simulink model "pid_analog_circuit"  (R2024b)
settings: Solver=ode4  StartTime=0.0  StopTime=1  FixedStep=pcb.sim_dt  RelTol=1e-3
PostLoadFcn:
  | pacdir_ = fileparts(get_param('pid_analog_circuit','FileName')); if ~exist('pcb','var'), run(fullfile(pacdir_,'pid_board_params.m')); end; if ~exist('pacirc','var'), run(fullfile(pacdir_,'pid_analog_circuit_params.m')); end; clear pacdir_
values from neighbouring files (symbols this model uses):
  pacirc = struct()    [pid_analog_circuit_params.m]
  pcb = evalin('base', 'pcb')    [pid_analog_circuit_test.m]    (also in pid_board_bench_inputs.m; pid_board_params.m = struct(); pid_board_validate.m)
libraries: ee_lib x153, fl_lib x61, nesl_utility x48
(part 1 of 5)
Description:
  | PID_Board rev B analog section, Simscape Electrical component-level model (circuit variant). Ports per ANALOG_INTERFACE.md. Params: pcb (pid_board_params.m) + pacirc (pid_analog_circuit_params.m).
settings Model: Creator=doubi  LastModifiedBy=doubi
settings DataIOCC: LoadExternalInput=on  SaveFormat=StructureWithTime

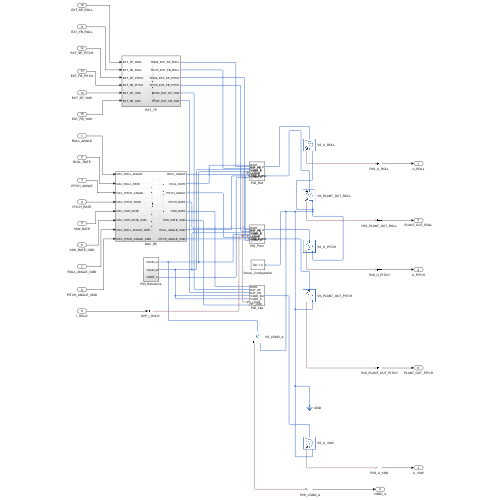
[thumbnail: Simulink's stored preview of the top-level diagram]
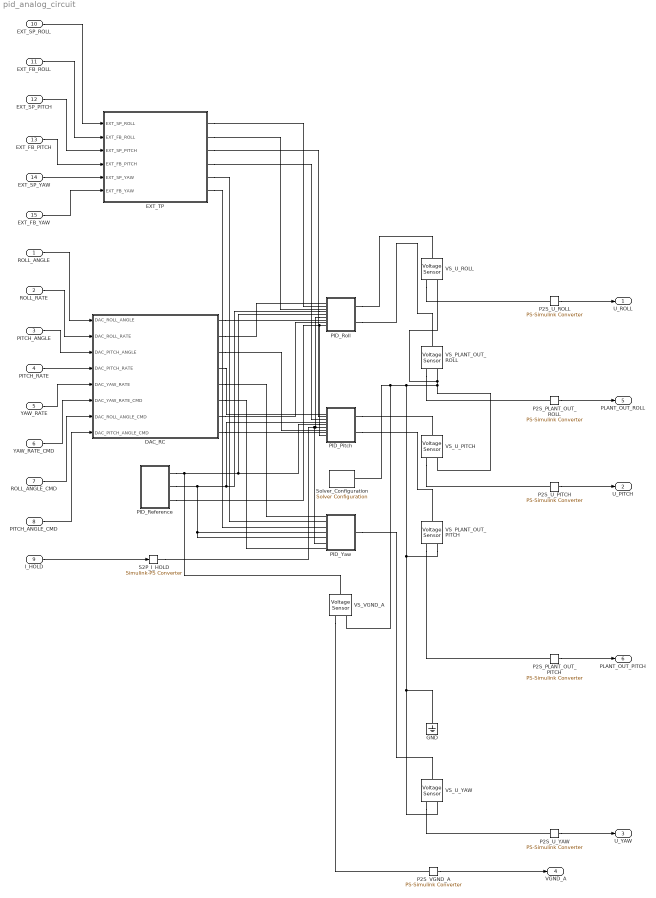
== system pid_analog_circuit ==
  ROLL_ANGLE : Inport
  ROLL_RATE : Inport  Port=2
  PITCH_ANGLE : Inport  Port=3
  PITCH_RATE : Inport  Port=4
  YAW_RATE : Inport  Port=5
  YAW_RATE_CMD : Inport  Port=6
  ROLL_ANGLE_CMD : Inport  Port=7
  PITCH_ANGLE_CMD : Inport  Port=8
  I_HOLD : Inport  Port=9
  EXT_SP_ROLL : Inport  Port=10
  EXT_FB_ROLL : Inport  Port=11
  EXT_SP_PITCH : Inport  Port=12
  EXT_FB_PITCH : Inport  Port=13
  EXT_SP_YAW : Inport  Port=14
  EXT_FB_YAW : Inport  Port=15
  DAC_RC : Subsystem
  EXT_TP : Subsystem
  GND : fl_lib/Electrical/Electrical Elements/Electrical Reference
  P2S_PLANT_OUT_PITCH : nesl_utility/PS-Simulink Converter  PhysicalDomain=network_engine_domain  SubClassName=ps_output  LeftPortType=input  RightPortType=output  PseudoPeriodic=off  Frequencies=[]  VectorFormat=inherit  Unit=V  AffineConversion=off
  P2S_PLANT_OUT_ROLL : nesl_utility/PS-Simulink Converter  PhysicalDomain=network_engine_domain  SubClassName=ps_output  LeftPortType=input  RightPortType=output  PseudoPeriodic=off  Frequencies=[]  VectorFormat=inherit  Unit=V  AffineConversion=off
  P2S_U_PITCH : nesl_utility/PS-Simulink Converter  PhysicalDomain=network_engine_domain  SubClassName=ps_output  LeftPortType=input  RightPortType=output  PseudoPeriodic=off  Frequencies=[]  VectorFormat=inherit  Unit=V  AffineConversion=off
  P2S_U_ROLL : nesl_utility/PS-Simulink Converter  PhysicalDomain=network_engine_domain  SubClassName=ps_output  LeftPortType=input  RightPortType=output  PseudoPeriodic=off  Frequencies=[]  VectorFormat=inherit  Unit=V  AffineConversion=off
  P2S_U_YAW : nesl_utility/PS-Simulink Converter  PhysicalDomain=network_engine_domain  SubClassName=ps_output  LeftPortType=input  RightPortType=output  PseudoPeriodic=off  Frequencies=[]  VectorFormat=inherit  Unit=V  AffineConversion=off
  P2S_VGND_A : nesl_utility/PS-Simulink Converter  PhysicalDomain=network_engine_domain  SubClassName=ps_output  LeftPortType=input  RightPortType=output  PseudoPeriodic=off  Frequencies=[]  VectorFormat=inherit  Unit=V  AffineConversion=off
  PID_Pitch : Subsystem  mask{ax=pcb.pitch}
      mask prompts: ax "Axis parameter struct (pcb.roll / pcb.pitch / pcb.yaw)"
      mask help: PID_Roll sheet (U201/U202, U9A): rate cell + angle loop + bench plant. Values from pcb.roll; part models from pacirc.
  PID_Reference : Subsystem
  PID_Roll : Subsystem  mask{ax=pcb.roll}
      mask prompts: ax "Axis parameter struct (pcb.roll / pcb.pitch / pcb.yaw)"
      mask help: PID_Roll sheet (U201/U202, U9A): rate cell + angle loop + bench plant. Values from pcb.roll; part models from pacirc.
  PID_Yaw : Subsystem  mask{ax=pcb.yaw}
      mask prompts: ax "Axis parameter struct (pcb.roll / pcb.pitch / pcb.yaw)"
      mask help: PID_Roll sheet (U201/U202, U9A): rate cell + angle loop + bench plant. Values from pcb.roll; part models from pacirc.
  S2P_I_HOLD : nesl_utility/Simulink-PS Converter  PhysicalDomain=network_engine_domain  SubClassName=ps_input  LeftPortType=input  RightPortType=output  PseudoPeriodic=off  Frequencies=[]  NoiseDistribution=none  NoiseParameters=[]  Unit=1  AffineConversion=off  FilteringAndDerivatives=provide  SimscapeFilterOrder=1  InputFilterTimeConstant=0.001  UdotUserProvided=0
  Solver_Configuration : nesl_utility/Solver Configuration  PhysicalDomain=network_engine_domain  SubClassName=solver  LeftPortType=input  RightPortType=generic  Tones=[]  Harmonics=[]  SimulateNoise=off  Profile=off  UseLocalSampling=off  EnableSwitchedLinearOptims=on  FrequencyDomain=off  UseCCode=off  RelTol=0.001  AbsTol=0.001  MinStep=1e-09  ToWorkspace=off  RevertToSquareIcSolve=off  NumHomotopyIterations=100  PhasorMode=off  PhasorModeNumHarmonics=1  ConsistencySolver=NEWTON_XTOL_AFTER_FTOL  IndexReductionMethod=DerivativeReplacement  DoDC=off  ResidualTolerance=1e-09  ConsistencyTolSource=GLOBAL  ConsistencyAbsTol=0.001  ConsistencyRelTol=0.001  ConsistencyTolFactor=0.001  UseLocalSolver=on  LocalSolverChoice=NE_BACKWARD_EULER_ADVANCER  ResolveIndetEquations=on  FunctionEvalNumThread=1  LocalSolverSampleTime=pacirc.Ts  DoFixedCost=on  MaxNonlinIter=pacirc.nl_iter  MaxModeIter=2  ComputeImpulses=off  ImpulseIterations=2  LinearAlgebra=auto  LinearAlgebraNumThread=0  EquationFormulation=NE_TIME_EF  DelaysMemoryBudget=1024  AutomaticFiltering=on  FilteringTimeConstant=0.001  PartitionStorageMethod=AS_NEEDED  PartitionMemoryBudget=1024  PartitionMethod=ROBUST  MultibodyUseLocalSolver=off  MultibodyLocalSolverChoice=ODE1  MultibodyLocalSolverSampleTime=0.001
  VS_PLANT_OUT_PITCH : fl_lib/Electrical/Electrical Sensors/Voltage Sensor
  VS_PLANT_OUT_ROLL : fl_lib/Electrical/Electrical Sensors/Voltage Sensor
  VS_U_PITCH : fl_lib/Electrical/Electrical Sensors/Voltage Sensor
  VS_U_ROLL : fl_lib/Electrical/Electrical Sensors/Voltage Sensor
  VS_U_YAW : fl_lib/Electrical/Electrical Sensors/Voltage Sensor
  VS_VGND_A : fl_lib/Electrical/Electrical Sensors/Voltage Sensor
  U_ROLL : Outport
  U_PITCH : Outport  Port=2
  U_YAW : Outport  Port=3
  VGND_A : Outport  Port=4
  PLANT_OUT_ROLL : Outport  Port=5
  PLANT_OUT_PITCH : Outport  Port=6
  wires:
  P2S_PLANT_OUT_PITCH/1 -> PLANT_OUT_PITCH/1
  P2S_PLANT_OUT_ROLL/1 -> PLANT_OUT_ROLL/1
  P2S_VGND_A/1 -> VGND_A/1
  P2S_U_YAW/1 -> U_YAW/1
  P2S_U_PITCH/1 -> U_PITCH/1
  P2S_U_ROLL/1 -> U_ROLL/1
  I_HOLD/1 -> S2P_I_HOLD/1
  EXT_FB_YAW/1 -> EXT_TP/6(EXT_FB_YAW)
  EXT_SP_YAW/1 -> EXT_TP/5(EXT_SP_YAW)
  EXT_FB_PITCH/1 -> EXT_TP/4(EXT_FB_PITCH)
  ROLL_ANGLE/1 -> DAC_RC/1(DAC_ROLL_ANGLE)
  ROLL_RATE/1 -> DAC_RC/2(DAC_ROLL_RATE)
  PITCH_ANGLE/1 -> DAC_RC/3(DAC_PITCH_ANGLE)
  PITCH_RATE/1 -> DAC_RC/4(DAC_PITCH_RATE)
  YAW_RATE/1 -> DAC_RC/5(DAC_YAW_RATE)
  YAW_RATE_CMD/1 -> DAC_RC/6(DAC_YAW_RATE_CMD)
  ROLL_ANGLE_CMD/1 -> DAC_RC/7(DAC_ROLL_ANGLE_CMD)
  PITCH_ANGLE_CMD/1 -> DAC_RC/8(DAC_PITCH_ANGLE_CMD)
  EXT_SP_ROLL/1 -> EXT_TP/1(EXT_SP_ROLL)
  EXT_FB_ROLL/1 -> EXT_TP/2(EXT_FB_ROLL)
  EXT_SP_PITCH/1 -> EXT_TP/3(EXT_SP_PITCH)
  connections:
  VS_PLANT_OUT_PITCH/RConn1 -- P2S_PLANT_OUT_PITCH/LConn1
  PID_Pitch/RConn2 -- VS_PLANT_OUT_PITCH/LConn1
  VS_PLANT_OUT_ROLL/RConn1 -- P2S_PLANT_OUT_ROLL/LConn1
  PID_Roll/RConn2 -- VS_PLANT_OUT_ROLL/LConn1
  VS_VGND_A/RConn1 -- P2S_VGND_A/LConn1
  VS_U_YAW/RConn1 -- P2S_U_YAW/LConn1
  PID_Yaw/RConn1 -- VS_U_YAW/LConn1
  VS_U_PITCH/RConn1 -- P2S_U_PITCH/LConn1
  PID_Pitch/RConn1 -- VS_U_PITCH/LConn1
  VS_U_ROLL/RConn1 -- P2S_U_ROLL/LConn1
  PID_Roll/RConn1 -- VS_U_ROLL/LConn1
  VS_PLANT_OUT_PITCH/RConn2 -- VS_U_YAW/RConn2 -- GND/LConn1 -- VS_VGND_A/RConn2 -- Solver_Configuration/RConn1 -- VS_PLANT_OUT_ROLL/RConn2 -- VS_U_ROLL/RConn2 -- VS_U_PITCH/RConn2
  EXT_TP/RConn6 -- PID_Yaw/LConn3
  EXT_TP/RConn5 -- PID_Yaw/LConn2
  EXT_TP/RConn4 -- PID_Pitch/LConn3
  EXT_TP/RConn3 -- PID_Pitch/LConn2
  EXT_TP/RConn2 -- PID_Roll/LConn3
  EXT_TP/RConn1 -- PID_Roll/LConn2
  DAC_RC/RConn8 -- PID_Pitch/LConn8
  DAC_RC/RConn7 -- PID_Roll/LConn8
  DAC_RC/RConn6 -- PID_Yaw/LConn7
  DAC_RC/RConn5 -- PID_Yaw/LConn1
  DAC_RC/RConn4 -- PID_Pitch/LConn1
  DAC_RC/RConn3 -- PID_Pitch/LConn7
  DAC_RC/RConn2 -- PID_Roll/LConn1
  DAC_RC/RConn1 -- PID_Roll/LConn7
  PID_Pitch/LConn9 -- PID_Reference/RConn3 -- PID_Roll/LConn9
  PID_Roll/LConn4 -- PID_Reference/RConn2 -- PID_Yaw/LConn4 -- PID_Yaw/LConn5 -- PID_Pitch/LConn4
  PID_Pitch/LConn5 -- PID_Reference/RConn1 -- VS_VGND_A/LConn1 -- PID_Roll/LConn5
  PID_Roll/LConn6 -- S2P_I_HOLD/RConn1 -- PID_Yaw/LConn6 -- PID_Pitch/LConn6

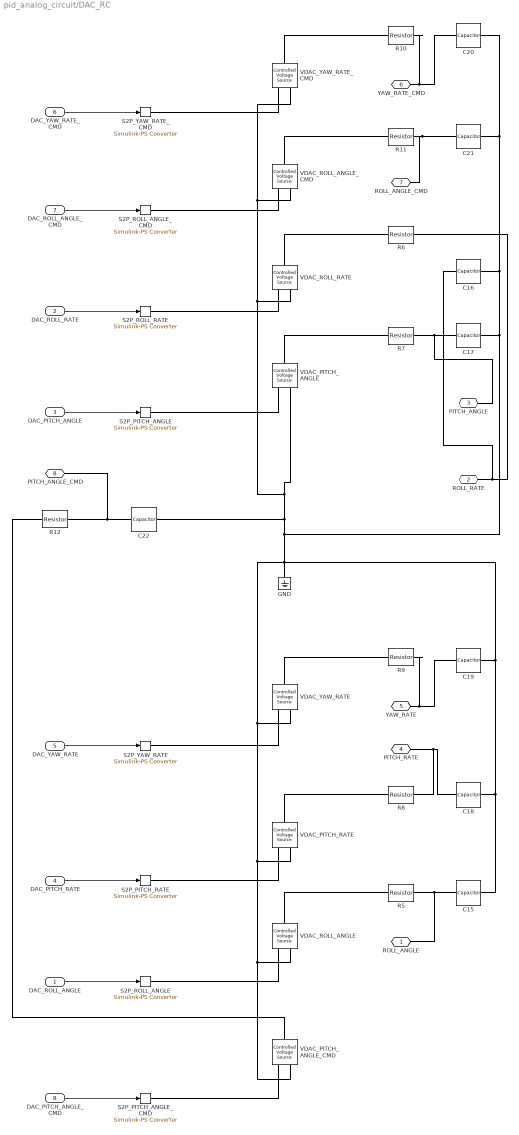
== system pid_analog_circuit/DAC_RC ==
  DAC_ROLL_ANGLE : Inport
  DAC_ROLL_RATE : Inport  Port=2
  DAC_PITCH_ANGLE : Inport  Port=3
  DAC_PITCH_RATE : Inport  Port=4
  DAC_YAW_RATE : Inport  Port=5
  DAC_YAW_RATE_CMD : Inport  Port=6
  DAC_ROLL_ANGLE_CMD : Inport  Port=7
  DAC_PITCH_ANGLE_CMD : Inport  Port=8
  C{15..22} (8 alike) : ee_lib/Passive/Capacitor  cap_option=ee.enum.passive.capacitor.capOption.const  c=pcb.dac.C_f F  Cvec=[1e-05, 1e-06] F  Vvec=[0, 10] V  CV_table_symmetry=ee.enum.passive.capacitor.tableSymmetry.yes  f_vec=[1, 10] kHz  DFext_vec=[.8, 1.2]  enable_C_tol=ee.enum.toleranceApplication.none  averaging_period=0 s  C_tol=5  tol_distribution=ee.enum.toleranceDistribution.uniform  nSigma=4  r=0 Ohm  g=0 1/Ohm  enable_operating_limits=ee.enum.enable.no  operating_limit_action=ee.enum.passive.reportOpLim.warn  max_working_voltage_range=[-25, 25] V  power_rating=1 W  maxTemperature=85 degC  thermalEnable=false  thermalMass=1 J/K  fault_action=simscape.enum.assert.action.none  t_fault=1 s  i_specify=off  i_priority=None  i=0 A  i_nominal_specify=off  i_nominal_value=1  i_nominal_unit=A  v_specify=off  v_priority=None  v=0 V  v_nominal_specify=off  v_nominal_value=1  v_nominal_unit=V  vc_specify=on  vc_priority=High  vc=pacirc.V0_dac V  vc_nominal_specify=off  vc_nominal_value=1  vc_nominal_unit=V  T_specify=off  T_priority=None  T=298.15 K  T_nominal_specify=off  T_nominal_value=1  T_nominal_unit=K
  GND : fl_lib/Electrical/Electrical Elements/Electrical Reference
  R10 : ee_lib/Passive/Resistor  R=pcb.dac.R_f Ohm  enable_R_tol=ee.enum.toleranceApplication.none  R_tol=5  tol_distribution=ee.enum.toleranceDistribution.uniform  nSigma=4  enable_operating_limits=ee.enum.enable.no  operating_limit_action=ee.enum.passive.reportOpLim.warn  power_rating=1 W  max_working_voltage=100 V  noise_mode=ee.enum.sources.noise.Disabled  Tdevice=25 degC  sample_time=1e-3 s  repeatability=ee.enum.ic.repeatability.notRepeatable  user_seed=0  auto_seed=1447930733  fault_action=simscape.enum.assert.action.none  t_fault=1 s  power_derating_T1=70 degC  power_derating_T2=155 degC  operating_temperature_range_vec=[-50, 150] degC  alpha=3.93e-3 1/K  Tmeas=25 degC  thermal_mass=100 J/K  temperature_specify=off  temperature_priority=High  temperature=298.15 K  temperature_nominal_specify=off  temperature_nominal_value=1  temperature_nominal_unit=K
  R11 : ee_lib/Passive/Resistor  R=pcb.dac.R_f Ohm  enable_R_tol=ee.enum.toleranceApplication.none  R_tol=5  tol_distribution=ee.enum.toleranceDistribution.uniform  nSigma=4  enable_operating_limits=ee.enum.enable.no  operating_limit_action=ee.enum.passive.reportOpLim.warn  power_rating=1 W  max_working_voltage=100 V  noise_mode=ee.enum.sources.noise.Disabled  Tdevice=25 degC  sample_time=1e-3 s  repeatability=ee.enum.ic.repeatability.notRepeatable  user_seed=0  auto_seed=696567710  fault_action=simscape.enum.assert.action.none  t_fault=1 s  power_derating_T1=70 degC  power_derating_T2=155 degC  operating_temperature_range_vec=[-50, 150] degC  alpha=3.93e-3 1/K  Tmeas=25 degC  thermal_mass=100 J/K  temperature_specify=off  temperature_priority=High  temperature=298.15 K  temperature_nominal_specify=off  temperature_nominal_value=1  temperature_nominal_unit=K
  R12 : ee_lib/Passive/Resistor  R=pcb.dac.R_f Ohm  enable_R_tol=ee.enum.toleranceApplication.none  R_tol=5  tol_distribution=ee.enum.toleranceDistribution.uniform  nSigma=4  enable_operating_limits=ee.enum.enable.no  operating_limit_action=ee.enum.passive.reportOpLim.warn  power_rating=1 W  max_working_voltage=100 V  noise_mode=ee.enum.sources.noise.Disabled  Tdevice=25 degC  sample_time=1e-3 s  repeatability=ee.enum.ic.repeatability.notRepeatable  user_seed=0  auto_seed=3411426126  fault_action=simscape.enum.assert.action.none  t_fault=1 s  power_derating_T1=70 degC  power_derating_T2=155 degC  operating_temperature_range_vec=[-50, 150] degC  alpha=3.93e-3 1/K  Tmeas=25 degC  thermal_mass=100 J/K  temperature_specify=off  temperature_priority=High  temperature=298.15 K  temperature_nominal_specify=off  temperature_nominal_value=1  temperature_nominal_unit=K
  R5 : ee_lib/Passive/Resistor  R=pcb.dac.R_f Ohm  enable_R_tol=ee.enum.toleranceApplication.none  R_tol=5  tol_distribution=ee.enum.toleranceDistribution.uniform  nSigma=4  enable_operating_limits=ee.enum.enable.no  operating_limit_action=ee.enum.passive.reportOpLim.warn  power_rating=1 W  max_working_voltage=100 V  noise_mode=ee.enum.sources.noise.Disabled  Tdevice=25 degC  sample_time=1e-3 s  repeatability=ee.enum.ic.repeatability.notRepeatable  user_seed=0  auto_seed=4011545342  fault_action=simscape.enum.assert.action.none  t_fault=1 s  power_derating_T1=70 degC  power_derating_T2=155 degC  operating_temperature_range_vec=[-50, 150] degC  alpha=3.93e-3 1/K  Tmeas=25 degC  thermal_mass=100 J/K  temperature_specify=off  temperature_priority=High  temperature=298.15 K  temperature_nominal_specify=off  temperature_nominal_value=1  temperature_nominal_unit=K
  R6 : ee_lib/Passive/Resistor  R=pcb.dac.R_f Ohm  enable_R_tol=ee.enum.toleranceApplication.none  R_tol=5  tol_distribution=ee.enum.toleranceDistribution.uniform  nSigma=4  enable_operating_limits=ee.enum.enable.no  operating_limit_action=ee.enum.passive.reportOpLim.warn  power_rating=1 W  max_working_voltage=100 V  noise_mode=ee.enum.sources.noise.Disabled  Tdevice=25 degC  sample_time=1e-3 s  repeatability=ee.enum.ic.repeatability.notRepeatable  user_seed=0  auto_seed=557942917  fault_action=simscape.enum.assert.action.none  t_fault=1 s  power_derating_T1=70 degC  power_derating_T2=155 degC  operating_temperature_range_vec=[-50, 150] degC  alpha=3.93e-3 1/K  Tmeas=25 degC  thermal_mass=100 J/K  temperature_specify=off  temperature_priority=High  temperature=298.15 K  temperature_nominal_specify=off  temperature_nominal_value=1  temperature_nominal_unit=K
  R7 : ee_lib/Passive/Resistor  R=pcb.dac.R_f Ohm  enable_R_tol=ee.enum.toleranceApplication.none  R_tol=5  tol_distribution=ee.enum.toleranceDistribution.uniform  nSigma=4  enable_operating_limits=ee.enum.enable.no  operating_limit_action=ee.enum.passive.reportOpLim.warn  power_rating=1 W  max_working_voltage=100 V  noise_mode=ee.enum.sources.noise.Disabled  Tdevice=25 degC  sample_time=1e-3 s  repeatability=ee.enum.ic.repeatability.notRepeatable  user_seed=0  auto_seed=2443079021  fault_action=simscape.enum.assert.action.none  t_fault=1 s  power_derating_T1=70 degC  power_derating_T2=155 degC  operating_temperature_range_vec=[-50, 150] degC  alpha=3.93e-3 1/K  Tmeas=25 degC  thermal_mass=100 J/K  temperature_specify=off  temperature_priority=High  temperature=298.15 K  temperature_nominal_specify=off  temperature_nominal_value=1  temperature_nominal_unit=K
  R8 : ee_lib/Passive/Resistor  R=pcb.dac.R_f Ohm  enable_R_tol=ee.enum.toleranceApplication.none  R_tol=5  tol_distribution=ee.enum.toleranceDistribution.uniform  nSigma=4  enable_operating_limits=ee.enum.enable.no  operating_limit_action=ee.enum.passive.reportOpLim.warn  power_rating=1 W  max_working_voltage=100 V  noise_mode=ee.enum.sources.noise.Disabled  Tdevice=25 degC  sample_time=1e-3 s  repeatability=ee.enum.ic.repeatability.notRepeatable  user_seed=0  auto_seed=2016017452  fault_action=simscape.enum.assert.action.none  t_fault=1 s  power_derating_T1=70 degC  power_derating_T2=155 degC  operating_temperature_range_vec=[-50, 150] degC  alpha=3.93e-3 1/K  Tmeas=25 degC  thermal_mass=100 J/K  temperature_specify=off  temperature_priority=High  temperature=298.15 K  temperature_nominal_specify=off  temperature_nominal_value=1  temperature_nominal_unit=K
  R9 : ee_lib/Passive/Resistor  R=pcb.dac.R_f Ohm  enable_R_tol=ee.enum.toleranceApplication.none  R_tol=5  tol_distribution=ee.enum.toleranceDistribution.uniform  nSigma=4  enable_operating_limits=ee.enum.enable.no  operating_limit_action=ee.enum.passive.reportOpLim.warn  power_rating=1 W  max_working_voltage=100 V  noise_mode=ee.enum.sources.noise.Disabled  Tdevice=25 degC  sample_time=1e-3 s  repeatability=ee.enum.ic.repeatability.notRepeatable  user_seed=0  auto_seed=51119000  fault_action=simscape.enum.assert.action.none  t_fault=1 s  power_derating_T1=70 degC  power_derating_T2=155 degC  operating_temperature_range_vec=[-50, 150] degC  alpha=3.93e-3 1/K  Tmeas=25 degC  thermal_mass=100 J/K  temperature_specify=off  temperature_priority=High  temperature=298.15 K  temperature_nominal_specify=off  temperature_nominal_value=1  temperature_nominal_unit=K
  S2P_PITCH_ANGLE : nesl_utility/Simulink-PS Converter  PhysicalDomain=network_engine_domain  SubClassName=ps_input  LeftPortType=input  RightPortType=output  PseudoPeriodic=off  Frequencies=[]  NoiseDistribution=none  NoiseParameters=[]  Unit=V  AffineConversion=off  FilteringAndDerivatives=provide  SimscapeFilterOrder=1  InputFilterTimeConstant=0.001  UdotUserProvided=0
  S2P_PITCH_ANGLE_CMD : nesl_utility/Simulink-PS Converter  PhysicalDomain=network_engine_domain  SubClassName=ps_input  LeftPortType=input  RightPortType=output  PseudoPeriodic=off  Frequencies=[]  NoiseDistribution=none  NoiseParameters=[]  Unit=V  AffineConversion=off  FilteringAndDerivatives=provide  SimscapeFilterOrder=1  InputFilterTimeConstant=0.001  UdotUserProvided=0
  S2P_PITCH_RATE : nesl_utility/Simulink-PS Converter  PhysicalDomain=network_engine_domain  SubClassName=ps_input  LeftPortType=input  RightPortType=output  PseudoPeriodic=off  Frequencies=[]  NoiseDistribution=none  NoiseParameters=[]  Unit=V  AffineConversion=off  FilteringAndDerivatives=provide  SimscapeFilterOrder=1  InputFilterTimeConstant=0.001  UdotUserProvided=0
  S2P_ROLL_ANGLE : nesl_utility/Simulink-PS Converter  PhysicalDomain=network_engine_domain  SubClassName=ps_input  LeftPortType=input  RightPortType=output  PseudoPeriodic=off  Frequencies=[]  NoiseDistribution=none  NoiseParameters=[]  Unit=V  AffineConversion=off  FilteringAndDerivatives=provide  SimscapeFilterOrder=1  InputFilterTimeConstant=0.001  UdotUserProvided=0
  S2P_ROLL_ANGLE_CMD : nesl_utility/Simulink-PS Converter  PhysicalDomain=network_engine_domain  SubClassName=ps_input  LeftPortType=input  RightPortType=output  PseudoPeriodic=off  Frequencies=[]  NoiseDistribution=none  NoiseParameters=[]  Unit=V  AffineConversion=off  FilteringAndDerivatives=provide  SimscapeFilterOrder=1  InputFilterTimeConstant=0.001  UdotUserProvided=0
  S2P_ROLL_RATE : nesl_utility/Simulink-PS Converter  PhysicalDomain=network_engine_domain  SubClassName=ps_input  LeftPortType=input  RightPortType=output  PseudoPeriodic=off  Frequencies=[]  NoiseDistribution=none  NoiseParameters=[]  Unit=V  AffineConversion=off  FilteringAndDerivatives=provide  SimscapeFilterOrder=1  InputFilterTimeConstant=0.001  UdotUserProvided=0
  S2P_YAW_RATE : nesl_utility/Simulink-PS Converter  PhysicalDomain=network_engine_domain  SubClassName=ps_input  LeftPortType=input  RightPortType=output  PseudoPeriodic=off  Frequencies=[]  NoiseDistribution=none  NoiseParameters=[]  Unit=V  AffineConversion=off  FilteringAndDerivatives=provide  SimscapeFilterOrder=1  InputFilterTimeConstant=0.001  UdotUserProvided=0
  S2P_YAW_RATE_CMD : nesl_utility/Simulink-PS Converter  PhysicalDomain=network_engine_domain  SubClassName=ps_input  LeftPortType=input  RightPortType=output  PseudoPeriodic=off  Frequencies=[]  NoiseDistribution=none  NoiseParameters=[]  Unit=V  AffineConversion=off  FilteringAndDerivatives=provide  SimscapeFilterOrder=1  InputFilterTimeConstant=0.001  UdotUserProvided=0
  VDAC_PITCH_ANGLE : fl_lib/Electrical/Electrical Sources/Controlled Voltage Source
  VDAC_PITCH_ANGLE_CMD : fl_lib/Electrical/Electrical Sources/Controlled Voltage Source
  VDAC_PITCH_RATE : fl_lib/Electrical/Electrical Sources/Controlled Voltage Source
  VDAC_ROLL_ANGLE : fl_lib/Electrical/Electrical Sources/Controlled Voltage Source
  VDAC_ROLL_ANGLE_CMD : fl_lib/Electrical/Electrical Sources/Controlled Voltage Source
  VDAC_ROLL_RATE : fl_lib/Electrical/Electrical Sources/Controlled Voltage Source
  VDAC_YAW_RATE : fl_lib/Electrical/Electrical Sources/Controlled Voltage Source
  VDAC_YAW_RATE_CMD : fl_lib/Electrical/Electrical Sources/Controlled Voltage Source
  ROLL_ANGLE : PMIOPort  Side=Right
  ROLL_RATE : PMIOPort  Port=2  Side=Right
  PITCH_ANGLE : PMIOPort  Port=3  Side=Right
  PITCH_RATE : PMIOPort  Port=4  Side=Right
  YAW_RATE : PMIOPort  Port=5  Side=Right
  YAW_RATE_CMD : PMIOPort  Port=6  Side=Right
  ROLL_ANGLE_CMD : PMIOPort  Port=7  Side=Right
  PITCH_ANGLE_CMD : PMIOPort  Port=8  Side=Right
  wires:
  DAC_PITCH_ANGLE_CMD/1 -> S2P_PITCH_ANGLE_CMD/1
  DAC_ROLL_ANGLE_CMD/1 -> S2P_ROLL_ANGLE_CMD/1
  DAC_YAW_RATE_CMD/1 -> S2P_YAW_RATE_CMD/1
  DAC_YAW_RATE/1 -> S2P_YAW_RATE/1
  DAC_PITCH_RATE/1 -> S2P_PITCH_RATE/1
  DAC_PITCH_ANGLE/1 -> S2P_PITCH_ANGLE/1
  DAC_ROLL_RATE/1 -> S2P_ROLL_RATE/1
  DAC_ROLL_ANGLE/1 -> S2P_ROLL_ANGLE/1
  connections:
  PITCH_ANGLE_CMD/RConn1 -- C22/LConn1 -- R12/RConn1
  VDAC_PITCH_ANGLE_CMD/LConn1 -- R12/LConn1
  S2P_PITCH_ANGLE_CMD/RConn1 -- VDAC_PITCH_ANGLE_CMD/RConn1
  ROLL_ANGLE_CMD/RConn1 -- R11/RConn1 -- C21/LConn1
  VDAC_ROLL_ANGLE_CMD/LConn1 -- R11/LConn1
  S2P_ROLL_ANGLE_CMD/RConn1 -- VDAC_ROLL_ANGLE_CMD/RConn1
  YAW_RATE_CMD/RConn1 -- R10/RConn1 -- C20/LConn1
  VDAC_YAW_RATE_CMD/LConn1 -- R10/LConn1
  S2P_YAW_RATE_CMD/RConn1 -- VDAC_YAW_RATE_CMD/RConn1
  YAW_RATE/RConn1 -- R9/RConn1 -- C19/LConn1
  VDAC_YAW_RATE/LConn1 -- R9/LConn1
  S2P_YAW_RATE/RConn1 -- VDAC_YAW_RATE/RConn1
  R8/RConn1 -- PITCH_RATE/RConn1 -- C18/LConn1
  VDAC_PITCH_RATE/LConn1 -- R8/LConn1
  S2P_PITCH_RATE/RConn1 -- VDAC_PITCH_RATE/RConn1
  PITCH_ANGLE/RConn1 -- R7/RConn1 -- C17/LConn1
  VDAC_PITCH_ANGLE/LConn1 -- R7/LConn1
  S2P_PITCH_ANGLE/RConn1 -- VDAC_PITCH_ANGLE/RConn1
  R6/RConn1 -- ROLL_RATE/RConn1 -- C16/LConn1
  VDAC_ROLL_RATE/LConn1 -- R6/LConn1
  S2P_ROLL_RATE/RConn1 -- VDAC_ROLL_RATE/RConn1
  ROLL_ANGLE/RConn1 -- C15/LConn1 -- R5/RConn1
  VDAC_ROLL_ANGLE/LConn1 -- R5/LConn1
  C18/RConn1 -- VDAC_PITCH_ANGLE_CMD/RConn2 -- VDAC_ROLL_ANGLE/RConn2 -- VDAC_PITCH_RATE/RConn2 -- VDAC_YAW_RATE/RConn2 -- C20/RConn1 -- C21/RConn1 -- C16/RConn1 -- C17/RConn1 -- VDAC_YAW_RATE_CMD/RConn2 -- VDAC_ROLL_ANGLE_CMD/RConn2 -- VDAC_ROLL_RATE/RConn2 -- VDAC_PITCH_ANGLE/RConn2 -- C22/RConn1 -- GND/LConn1 -- C19/RConn1 -- C15/RConn1
  S2P_ROLL_ANGLE/RConn1 -- VDAC_ROLL_ANGLE/RConn1

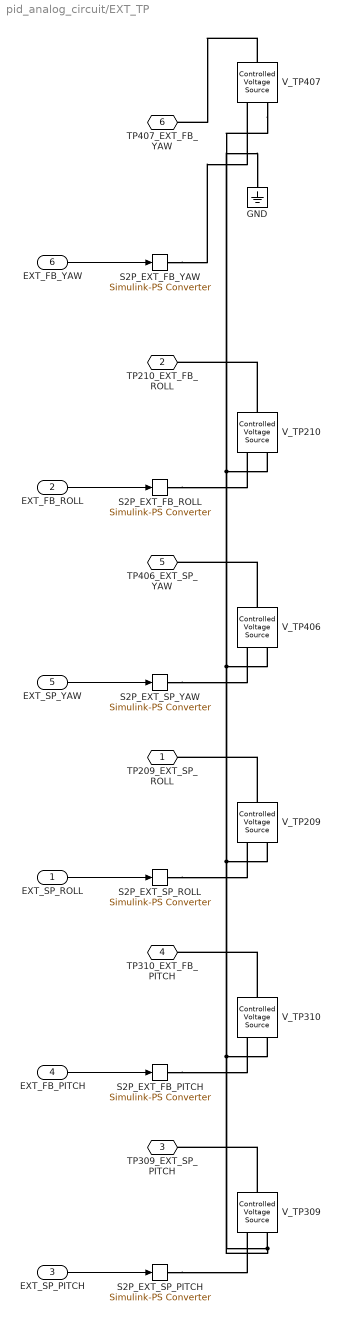
== system pid_analog_circuit/EXT_TP ==
  EXT_SP_ROLL : Inport
  EXT_FB_ROLL : Inport  Port=2
  EXT_SP_PITCH : Inport  Port=3
  EXT_FB_PITCH : Inport  Port=4
  EXT_SP_YAW : Inport  Port=5
  EXT_FB_YAW : Inport  Port=6
  GND : fl_lib/Electrical/Electrical Elements/Electrical Reference
  S2P_EXT_FB_PITCH : nesl_utility/Simulink-PS Converter  PhysicalDomain=network_engine_domain  SubClassName=ps_input  LeftPortType=input  RightPortType=output  PseudoPeriodic=off  Frequencies=[]  NoiseDistribution=none  NoiseParameters=[]  Unit=V  AffineConversion=off  FilteringAndDerivatives=provide  SimscapeFilterOrder=1  InputFilterTimeConstant=0.001  UdotUserProvided=0
  S2P_EXT_FB_ROLL : nesl_utility/Simulink-PS Converter  PhysicalDomain=network_engine_domain  SubClassName=ps_input  LeftPortType=input  RightPortType=output  PseudoPeriodic=off  Frequencies=[]  NoiseDistribution=none  NoiseParameters=[]  Unit=V  AffineConversion=off  FilteringAndDerivatives=provide  SimscapeFilterOrder=1  InputFilterTimeConstant=0.001  UdotUserProvided=0
  S2P_EXT_FB_YAW : nesl_utility/Simulink-PS Converter  PhysicalDomain=network_engine_domain  SubClassName=ps_input  LeftPortType=input  RightPortType=output  PseudoPeriodic=off  Frequencies=[]  NoiseDistribution=none  NoiseParameters=[]  Unit=V  AffineConversion=off  FilteringAndDerivatives=provide  SimscapeFilterOrder=1  InputFilterTimeConstant=0.001  UdotUserProvided=0
  S2P_EXT_SP_PITCH : nesl_utility/Simulink-PS Converter  PhysicalDomain=network_engine_domain  SubClassName=ps_input  LeftPortType=input  RightPortType=output  PseudoPeriodic=off  Frequencies=[]  NoiseDistribution=none  NoiseParameters=[]  Unit=V  AffineConversion=off  FilteringAndDerivatives=provide  SimscapeFilterOrder=1  InputFilterTimeConstant=0.001  UdotUserProvided=0
  S2P_EXT_SP_ROLL : nesl_utility/Simulink-PS Converter  PhysicalDomain=network_engine_domain  SubClassName=ps_input  LeftPortType=input  RightPortType=output  PseudoPeriodic=off  Frequencies=[]  NoiseDistribution=none  NoiseParameters=[]  Unit=V  AffineConversion=off  FilteringAndDerivatives=provide  SimscapeFilterOrder=1  InputFilterTimeConstant=0.001  UdotUserProvided=0
  S2P_EXT_SP_YAW : nesl_utility/Simulink-PS Converter  PhysicalDomain=network_engine_domain  SubClassName=ps_input  LeftPortType=input  RightPortType=output  PseudoPeriodic=off  Frequencies=[]  NoiseDistribution=none  NoiseParameters=[]  Unit=V  AffineConversion=off  FilteringAndDerivatives=provide  SimscapeFilterOrder=1  InputFilterTimeConstant=0.001  UdotUserProvided=0
  V_TP{209..210,309..310,406..407} (6 alike) : fl_lib/Electrical/Electrical Sources/Controlled Voltage Source
  TP209_EXT_SP_ROLL : PMIOPort  Side=Right
  TP210_EXT_FB_ROLL : PMIOPort  Port=2  Side=Right
  TP309_EXT_SP_PITCH : PMIOPort  Port=3  Side=Right
  TP310_EXT_FB_PITCH : PMIOPort  Port=4  Side=Right
  TP406_EXT_SP_YAW : PMIOPort  Port=5  Side=Right
  TP407_EXT_FB_YAW : PMIOPort  Port=6  Side=Right
  wires:
  EXT_FB_YAW/1 -> S2P_EXT_FB_YAW/1
  EXT_SP_YAW/1 -> S2P_EXT_SP_YAW/1
  EXT_FB_PITCH/1 -> S2P_EXT_FB_PITCH/1
  EXT_SP_PITCH/1 -> S2P_EXT_SP_PITCH/1
  EXT_FB_ROLL/1 -> S2P_EXT_FB_ROLL/1
  EXT_SP_ROLL/1 -> S2P_EXT_SP_ROLL/1
  connections:
  V_TP407/LConn1 -- TP407_EXT_FB_YAW/RConn1
  S2P_EXT_FB_YAW/RConn1 -- V_TP407/RConn1
  V_TP406/LConn1 -- TP406_EXT_SP_YAW/RConn1
  S2P_EXT_SP_YAW/RConn1 -- V_TP406/RConn1
  V_TP310/LConn1 -- TP310_EXT_FB_PITCH/RConn1
  S2P_EXT_FB_PITCH/RConn1 -- V_TP310/RConn1
  V_TP309/LConn1 -- TP309_EXT_SP_PITCH/RConn1
  S2P_EXT_SP_PITCH/RConn1 -- V_TP309/RConn1
  V_TP210/LConn1 -- TP210_EXT_FB_ROLL/RConn1
  S2P_EXT_FB_ROLL/RConn1 -- V_TP210/RConn1
  V_TP209/LConn1 -- TP209_EXT_SP_ROLL/RConn1
  V_TP407/RConn2 -- V_TP210/RConn2 -- GND/LConn1 -- V_TP406/RConn2 -- V_TP209/RConn2 -- V_TP310/RConn2 -- V_TP309/RConn2
  S2P_EXT_SP_ROLL/RConn1 -- V_TP209/RConn1
